simulink model "WT_FFNN_trainbfg_15_15_15_Dec_22_RepFast"  (R2021a)
settings: Solver=FixedStepAuto  StartTime=0  StopTime=T  FixedStep=Ts  RelTol=1e-3  EnableMultiTasking=on
undefined symbols (not defined in the file): patch_sig, safe_patch_sig, sw
libraries: neural x50, simulink x3
(part 2 of 2)

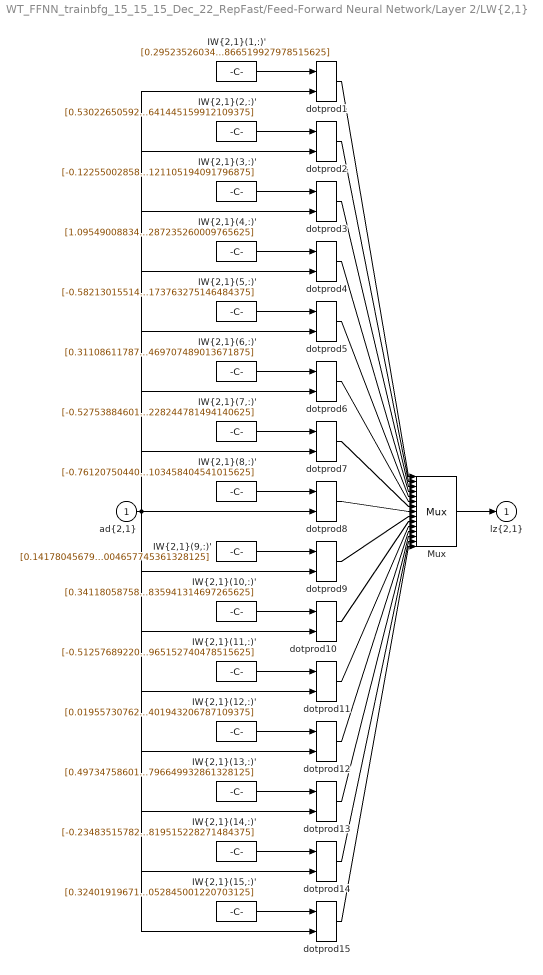
== system WT_FFNN_trainbfg_15_15_15_Dec_22_RepFast/Feed-Forward Neural Network/Layer 2/LW{2,1} ==
  "ad{2,1}" : Inport  PortDimensions=15
      mask Display: e = 0.06;c1 = [120 230 180]/255;c2 = ([120 230 180]+0)/(256+128);c3 = ([120 230 180]+128)/(256+128);patch([0 1 1 0],[0 0 1 1],c1);patch([0 1 1 1-e 1-e 0+e],[0 0 1 1-e 0+e 0+e],c2);patch([0 0 1 1-e 0+e 0+e],[0 1 1 1-e 1-e 0+e],c3);plot([0 1 1 0 0],[0 0 1 1 0]);
  "IW{2,1}(1,:)'" : Constant  Value=[0.295235260345368732970428027329035103321075439453125;-0.1676828200604070229218223175848834216594696044921875;0.089432221053525662313177235773764550685882568359375;0.54396077110849017088867185520939528942108154296875;-0.30457465744494971460198939894326031208038330078125;-0.96084475289336257475270031136460602283477783203125;0.5808144359338267559422774866106919944286346435546875;-0.1860903257221864226522711760480888187885284423828125;0.7014253485780148622552587767131626605987548828125;-0.54431412858791627940036050858907401561737060546875;0.5380581706717924017624454791075550019741058349609375;-0.9009348419158775822523921306128613650798797607421875;-0.7521354448038597428904949993011541664600372314453125;0.241917287870616615208518851432017982006072998046875;-0.7321374980240575869316899115801788866519927978515625]
      mask Display: e = 0.06;c1 = [120 150 230]/255;c2 = ([120 150 230]+0)/383;c3 = ([120 150 230]+128)/383;patch([0 1 1 0],[0 0 1 1],c1);patch([0 1 1 1-e 1-e 0+e],[0 0 1 1-e 0+e 0+e],c2);patch([0 0 1 1-e 0+e 0+e],[0 1 1 1-e 1-e 0+e],c3);plot([0 1 1 0 0],[0 0 1 1 0]);disp('weights');
  "IW{2,1}(10,:)'" : Constant  Value=[0.3411805875894959871885703250882215797901153564453125;-0.36412192595956416329983085233834572136402130126953125;-0.64636339290746036567725241184234619140625;0.722279622786664798894662453676573932170867919921875;-0.27904982791519883367215015823603607714176177978515625;0.68360886979400292684516671215533278882503509521484375;0.97808482860116885415635579192894510924816131591796875;0.6199190595393042624294821507646702229976654052734375;0.72843908277886437740988867517444305121898651123046875;-0.83326035111029117530279108905233442783355712890625;-0.58147330032467425819930895158904604613780975341796875;-0.30410030612850647013800653439830057322978973388671875;-0.58836623426168210837516880928887985646724700927734375;0.968838908437390955441514961421489715576171875;0.68377280483594038429373540566302835941314697265625]
      mask Display: e = 0.06;c1 = [120 150 230]/255;c2 = ([120 150 230]+0)/383;c3 = ([120 150 230]+128)/383;patch([0 1 1 0],[0 0 1 1],c1);patch([0 1 1 1-e 1-e 0+e],[0 0 1 1-e 0+e 0+e],c2);patch([0 0 1 1-e 0+e 0+e],[0 1 1 1-e 1-e 0+e],c3);plot([0 1 1 0 0],[0 0 1 1 0]);disp('weights');
  "IW{2,1}(11,:)'" : Constant  Value=[-0.512576892202383671559573485865257680416107177734375;-0.64166672849162242897591568180359899997711181640625;-0.2323014726512367678079584720762795768678188323974609375;-0.004885732283956631914756396639631930156610906124114990234375;0.66589137226295747051807438765536062419414520263671875;-0.2068744392450924396431588547784485854208469390869140625;0.055562400254155118461962814535581856034696102142333984375;-0.0276621328029923348179597297757936757989227771759033203125;0.22700116851777263349276836379431188106536865234375;0.381837877655510082863798970720381475985050201416015625;0.373687162446426024420276235105120576918125152587890625;0.10188044464799216048955798896713531576097011566162109375;0.928861560137871578035628772340714931488037109375;0.83619474780461811036502695060335099697113037109375;0.42233175405663969659286749447346664965152740478515625]
      mask Display: e = 0.06;c1 = [120 150 230]/255;c2 = ([120 150 230]+0)/383;c3 = ([120 150 230]+128)/383;patch([0 1 1 0],[0 0 1 1],c1);patch([0 1 1 1-e 1-e 0+e],[0 0 1 1-e 0+e 0+e],c2);patch([0 0 1 1-e 0+e 0+e],[0 1 1 1-e 1-e 0+e],c3);plot([0 1 1 0 0],[0 0 1 1 0]);disp('weights');
  "IW{2,1}(12,:)'" : Constant  Value=[0.0195573076253098519783346631584208807907998561859130859375;0.96877950329973661069971058168448507785797119140625;-0.43906894185078815251443984379875473678112030029296875;-0.2453583760887959874796848680489347316324710845947265625;-0.429912780674979233541677103858091868460178375244140625;0.454767949982676278342097475615446455776691436767578125;0.612974659896225571031891377060674130916595458984375;-0.784699422493088771801694747409783303737640380859375;0.97821339088929182281617613625712692737579345703125;0.422244862396419839978278787384624592959880828857421875;0.1638567334025056165813793995766900479793548583984375;0.1225489164995739732599844273863709531724452972412109375;-0.7051550721363504248273557095672003924846649169921875;0.39408876509436707724631787641556002199649810791015625;0.712830466285756525479655465460382401943206787109375]
      mask Display: e = 0.06;c1 = [120 150 230]/255;c2 = ([120 150 230]+0)/383;c3 = ([120 150 230]+128)/383;patch([0 1 1 0],[0 0 1 1],c1);patch([0 1 1 1-e 1-e 0+e],[0 0 1 1-e 0+e 0+e],c2);patch([0 0 1 1-e 0+e 0+e],[0 1 1 1-e 1-e 0+e],c3);plot([0 1 1 0 0],[0 0 1 1 0]);disp('weights');
  "IW{2,1}(13,:)'" : Constant  Value=[0.49734758601192741167551503167487680912017822265625;0.456087717212201482208655534122954122722148895263671875;-0.354850716647025776762092164062778465449810028076171875;0.370056821822693116086355757943238131701946258544921875;0.35945755073370933008192196211894042789936065673828125;0.403962590618102412864942607484408654272556304931640625;0.2812584438426630750740287112421356141567230224609375;0.01267604058140091478901201327289527398534119129180908203125;0.0501638531721098901439148676217882893979549407958984375;0.66191317537370519819006631223601289093494415283203125;-0.819786337588402691523015164420939981937408447265625;-0.0870564870349785635550432516538421623408794403076171875;-0.77059092798831418935634474109974689781665802001953125;0.06492564894049072943271738722614827565848827362060546875;-0.31005397435624815205557069930364377796649932861328125]
      mask Display: e = 0.06;c1 = [120 150 230]/255;c2 = ([120 150 230]+0)/383;c3 = ([120 150 230]+128)/383;patch([0 1 1 0],[0 0 1 1],c1);patch([0 1 1 1-e 1-e 0+e],[0 0 1 1-e 0+e 0+e],c2);patch([0 0 1 1-e 0+e 0+e],[0 1 1 1-e 1-e 0+e],c3);plot([0 1 1 0 0],[0 0 1 1 0]);disp('weights');
  "IW{2,1}(14,:)'" : Constant  Value=[-0.2348351578285707841331486633862368762493133544921875;-0.064245850300208129368684240034781396389007568359375;0.6412050242524041099301257418119348585605621337890625;0.483055790205989155072785479205776937305927276611328125;0.400497833477529485701751355009037069976329803466796875;-0.245029018628923456191159857553429901599884033203125;-0.69720340711643780107209522611810825765132904052734375;-0.70745219481255927629348434493294917047023773193359375;-0.040138572521909075818680179281727760098874568939208984375;0.78407918172274826407175396525417454540729522705078125;0.242397800141408048535396346778725273907184600830078125;0.07763798805447734430185136034197057597339153289794921875;-0.7345468453233909844612981032696552574634552001953125;-0.54799275931600222033779346020310185849666595458984375;-0.09452344436802194438396185205419897101819515228271484375]
      mask Display: e = 0.06;c1 = [120 150 230]/255;c2 = ([120 150 230]+0)/383;c3 = ([120 150 230]+128)/383;patch([0 1 1 0],[0 0 1 1],c1);patch([0 1 1 1-e 1-e 0+e],[0 0 1 1-e 0+e 0+e],c2);patch([0 0 1 1-e 0+e 0+e],[0 1 1 1-e 1-e 0+e],c3);plot([0 1 1 0 0],[0 0 1 1 0]);disp('weights');
  "IW{2,1}(15,:)'" : Constant  Value=[0.32401919671826906466094442293979227542877197265625;0.27772538922407574712991618071100674569606781005859375;0.25589672598047841223234399876673705875873565673828125;0.03997845702521808652907253645025775767862796783447265625;-0.116249832056752155917678237528889440000057220458984375;-0.56796216807721133790209933067671954631805419921875;-0.60041201485130313297844395492575131356716156005859375;-0.890051706187623636878925026394426822662353515625;0.60263542093203981142579550578375346958637237548828125;0.963512604604961353516046074219048023223876953125;-0.276048475872037124556612752712680958211421966552734375;-0.1097733012448873779476343770511448383331298828125;-0.66715673418933019167553766237688250839710235595703125;-0.2029144931375184424116042691821348853409290313720703125;-0.8924339193614028165058016384136863052845001220703125]
      mask Display: e = 0.06;c1 = [120 150 230]/255;c2 = ([120 150 230]+0)/383;c3 = ([120 150 230]+128)/383;patch([0 1 1 0],[0 0 1 1],c1);patch([0 1 1 1-e 1-e 0+e],[0 0 1 1-e 0+e 0+e],c2);patch([0 0 1 1-e 0+e 0+e],[0 1 1 1-e 1-e 0+e],c3);plot([0 1 1 0 0],[0 0 1 1 0]);disp('weights');
  "IW{2,1}(2,:)'" : Constant  Value=[0.5302265059205459873936661097104661166667938232421875;0.56475845138696723068960636737756431102752685546875;0.289664279816221614805016315585817210376262664794921875;0.8636390282028738596409311867319047451019287109375;-0.83362192000415868964324772605323232710361480712890625;-0.32183369212487911159570330710266716778278350830078125;0.75628015692548478110524001749581657350063323974609375;0.50230327800125673665121439626091159880161285400390625;0.11937217688658485759134464387898333370685577392578125;-0.09668324036885701799892700591954053379595279693603515625;-0.046385487394211201428451118999873870052397251129150390625;0.044395647902648216476251263884478248655796051025390625;-0.00954028462260186373156134465034483582712709903717041015625;0.03576122102860723739325976566760800778865814208984375;-1.087387383095764104012914685881696641445159912109375]
      mask Display: e = 0.06;c1 = [120 150 230]/255;c2 = ([120 150 230]+0)/383;c3 = ([120 150 230]+128)/383;patch([0 1 1 0],[0 0 1 1],c1);patch([0 1 1 1-e 1-e 0+e],[0 0 1 1-e 0+e 0+e],c2);patch([0 0 1 1-e 0+e 0+e],[0 1 1 1-e 1-e 0+e],c3);plot([0 1 1 0 0],[0 0 1 1 0]);disp('weights');
  "IW{2,1}(3,:)'" : Constant  Value=[-0.122550028588137294160986812130431644618511199951171875;0.8040681415155563893648604789632372558116912841796875;0.0700803874628591894069273848799639381468296051025390625;0.86939028804827123142473510597483254969120025634765625;0.412087729344845887791137784006423316895961761474609375;-0.29275208488329063083455139349098317325115203857421875;-0.421436955168346505384846523156738840043544769287109375;0.40171474062549805683630665953387506306171417236328125;0.86673742143877918753247513450332917273044586181640625;0.7464565387159451947951538386405445635318756103515625;0.77358975929442330699004060079460032284259796142578125;-0.74128481048777583595210671774111688137054443359375;1.0107702803741853703201059033744968473911285400390625;-1.015420261737861817863404212403111159801483154296875;0.99610375682476604008996901029604487121105194091796875]
      mask Display: e = 0.06;c1 = [120 150 230]/255;c2 = ([120 150 230]+0)/383;c3 = ([120 150 230]+128)/383;patch([0 1 1 0],[0 0 1 1],c1);patch([0 1 1 1-e 1-e 0+e],[0 0 1 1-e 0+e 0+e],c2);patch([0 0 1 1-e 0+e 0+e],[0 1 1 1-e 1-e 0+e],c3);plot([0 1 1 0 0],[0 0 1 1 0]);disp('weights');
  "IW{2,1}(4,:)'" : Constant  Value=[1.0954900883453830839897591431508772075176239013671875;-1.0671398314434192844402105038170702755451202392578125;0.4674545926284678909468084384570829570293426513671875;-0.622334117614310233790320125990547239780426025390625;-0.50044651341551193990397905508871190249919891357421875;-0.41617167669077270719668604215257801115512847900390625;0.554605315996658188026913194335065782070159912109375;0.68495334159006715513129393002600409090518951416015625;0.380392781972371418763856354416930116713047027587890625;-0.403210535716429119279524684316129423677921295166015625;0.0996010326827965475349202506549772806465625762939453125;-0.55362973136024018483425379599793814122676849365234375;0.76341803366177474199361085993587039411067962646484375;0.75787617513104288402558950110687874257564544677734375;-0.63575117538482450729730999228195287287235260009765625]
      mask Display: e = 0.06;c1 = [120 150 230]/255;c2 = ([120 150 230]+0)/383;c3 = ([120 150 230]+128)/383;patch([0 1 1 0],[0 0 1 1],c1);patch([0 1 1 1-e 1-e 0+e],[0 0 1 1-e 0+e 0+e],c2);patch([0 0 1 1-e 0+e 0+e],[0 1 1 1-e 1-e 0+e],c3);plot([0 1 1 0 0],[0 0 1 1 0]);disp('weights');
  "IW{2,1}(5,:)'" : Constant  Value=[-0.582130155147954297945034340955317020416259765625;0.226921473625750547142843061010353267192840576171875;0.0449906115542042517319032413070090115070343017578125;-0.7222515943416893957618185595492832362651824951171875;-0.9110918154435230231769082820392213761806488037109375;-0.6058924038090884867102658972726203501224517822265625;-0.122710034826088776327424056944437325000762939453125;-0.3629515092020156874497160970349796116352081298828125;0.165581930351680117752266596653498709201812744140625;0.6903563701080732695203323601162992417812347412109375;-0.96603412332547744512112330994568765163421630859375;-0.5890116581846402965538800344802439212799072265625;-0.45941133541460477118789640371687710285186767578125;0.457323363356542333946208600536920130252838134765625;-0.408932331049287167701322687207721173763275146484375]
      mask Display: e = 0.06;c1 = [120 150 230]/255;c2 = ([120 150 230]+0)/383;c3 = ([120 150 230]+128)/383;patch([0 1 1 0],[0 0 1 1],c1);patch([0 1 1 1-e 1-e 0+e],[0 0 1 1-e 0+e 0+e],c2);patch([0 0 1 1-e 0+e 0+e],[0 1 1 1-e 1-e 0+e],c3);plot([0 1 1 0 0],[0 0 1 1 0]);disp('weights');
  "IW{2,1}(6,:)'" : Constant  Value=[0.3110861178764547929631589795462787151336669921875;-0.538125541393581929838774158270098268985748291015625;1.0922620681325267977257453821948729455471038818359375;0.47206045307648636377706452549318782985210418701171875;0.406596366182418955670385685152723453938961029052734375;0.64098472753113833189075876362039707601070404052734375;0.69478739666693722920598474956932477653026580810546875;0.054751583517420716884505083044132334180176258087158203125;0.62813081168441431412219344565528444945812225341796875;-0.2061992856573582333368221952696330845355987548828125;-0.85292749069341422529788587780785746872425079345703125;-0.64614216631411014457597730142879299819469451904296875;-0.705984380169617953271199439768679440021514892578125;0.70665367079108165615508596602012403309345245361328125;-0.52734700314943949717161331136594526469707489013671875]
      mask Display: e = 0.06;c1 = [120 150 230]/255;c2 = ([120 150 230]+0)/383;c3 = ([120 150 230]+128)/383;patch([0 1 1 0],[0 0 1 1],c1);patch([0 1 1 1-e 1-e 0+e],[0 0 1 1-e 0+e 0+e],c2);patch([0 0 1 1-e 0+e 0+e],[0 1 1 1-e 1-e 0+e],c3);plot([0 1 1 0 0],[0 0 1 1 0]);disp('weights');
  "IW{2,1}(7,:)'" : Constant  Value=[-0.5275388460124068590317847338155843317508697509765625;0.63968120217193635834718179467017762362957000732421875;-1.4284826471654101798236524700769223272800445556640625;-0.87089994099444234532114705871208570897579193115234375;-0.727791167771064895219979007379151880741119384765625;-0.140157181233467209580112466937862336635589599609375;0.36231999642735213118527326514595188200473785400390625;-0.82009864245883790090374532155692577362060546875;0.75357372007314304962477535809739492833614349365234375;0.6501208183024740350219872198067605495452880859375;0.722174859333458929455673569464124739170074462890625;-0.78697167378918475577620483818463981151580810546875;0.469890026516892100882927252314402721822261810302734375;-1.1508080217275782342056800189311616122722625732421875;0.2368252313630880012684798430200316943228244781494140625]
      mask Display: e = 0.06;c1 = [120 150 230]/255;c2 = ([120 150 230]+0)/383;c3 = ([120 150 230]+128)/383;patch([0 1 1 0],[0 0 1 1],c1);patch([0 1 1 1-e 1-e 0+e],[0 0 1 1-e 0+e 0+e],c2);patch([0 0 1 1-e 0+e 0+e],[0 1 1 1-e 1-e 0+e],c3);plot([0 1 1 0 0],[0 0 1 1 0]);disp('weights');
  "IW{2,1}(8,:)'" : Constant  Value=[-0.7612075044053889794071210417314432561397552490234375;0.90690656912513512022400163914426229894161224365234375;-0.85143144253750058236818176737870089709758758544921875;0.04780801927375631643624132038894458673894405364990234375;-0.1744673941545842599243343329362687654793262481689453125;0.7755419085127075451424616403528489172458648681640625;-0.67686592553680269279681169791729189455509185791015625;-0.776588511613593102111963162315078079700469970703125;0.97930676436914365634578416575095616281032562255859375;-0.265526583954380723806565356426290236413478851318359375;-0.0072625998806437851162964847162584192119538784027099609375;-0.93420966482242018269488426085445098578929901123046875;0.1878646683548915452544036952531314454972743988037109375;0.7518711623440605951174120491486974060535430908203125;0.266611480614983575865295506446273066103458404541015625]
      mask Display: e = 0.06;c1 = [120 150 230]/255;c2 = ([120 150 230]+0)/383;c3 = ([120 150 230]+128)/383;patch([0 1 1 0],[0 0 1 1],c1);patch([0 1 1 1-e 1-e 0+e],[0 0 1 1-e 0+e 0+e],c2);patch([0 0 1 1-e 0+e 0+e],[0 1 1 1-e 1-e 0+e],c3);plot([0 1 1 0 0],[0 0 1 1 0]);disp('weights');
  "IW{2,1}(9,:)'" : Constant  Value=[0.1417804567956018058083600408281199634075164794921875;-0.69552074345356695861397611224674619734287261962890625;-0.8666039658670074974367025788524188101291656494140625;-0.01732820083515733411427817145522567443549633026123046875;0.2389862039024584217106195183077943511307239532470703125;-0.236256188189785609754522965886280871927738189697265625;0.63365984517294438038703674465068615972995758056640625;-0.76292736525968740668446343988762237131595611572265625;-1.0008999859346239258428568064118735492229461669921875;0.056428107179615917543546999013415188528597354888916015625;0.4593302753053769560409591576899401843547821044921875;0.2149457557622795611518284886187757365405559539794921875;-0.056642227092704888757879189142840914428234100341796875;0.63895629042777668527008927412680350244045257568359375;-1.008264007948838969497273865272291004657745361328125]
      mask Display: e = 0.06;c1 = [120 150 230]/255;c2 = ([120 150 230]+0)/383;c3 = ([120 150 230]+128)/383;patch([0 1 1 0],[0 0 1 1],c1);patch([0 1 1 1-e 1-e 0+e],[0 0 1 1-e 0+e 0+e],c2);patch([0 0 1 1-e 0+e 0+e],[0 1 1 1-e 1-e 0+e],c3);plot([0 1 1 0 0],[0 0 1 1 0]);disp('weights');
  Mux : Mux  Inputs=15
      mask Display: e = 0.06;c1 = [120 150 230]/255;c2 = ([120 150 230]+0)/383;c3 = ([120 150 230]+128)/383;patch([0 1 1 0],[0 0 1 1],c1);patch([0 1 1 1-e 1-e 0+e],[0 0 1 1-e 0+e 0+e],c2);patch([0 0 1 1-e 0+e 0+e],[0 1 1 1-e 1-e 0+e],c3);plot([0 1 1 0 0],[0 0 1 1 0]);disp('Mux');
  dotprod{1..15} (15 alike) : neural/Weight Functions/dotprod
  "lz{2,1}" : Outport
      mask Display: e = 0.06;c1 = [120 230 180]/255;c2 = ([120 230 180]+0)/(256+128);c3 = ([120 230 180]+128)/(256+128);patch([0 1 1 0],[0 0 1 1],c1);patch([0 1 1 1-e 1-e 0+e],[0 0 1 1-e 0+e 0+e],c2);patch([0 0 1 1-e 0+e 0+e],[0 1 1 1-e 1-e 0+e],c3);plot([0 1 1 0 0],[0 0 1 1 0]);
  wires:
  "IW{2,1}(1,:)'"/1 -> dotprod1/1
  "ad{2,1}"/1 -> dotprod1/2, dotprod2/2, dotprod3/2, dotprod4/2, dotprod5/2, dotprod6/2, dotprod7/2, dotprod8/2, dotprod9/2, dotprod10/2, dotprod11/2, dotprod12/2, dotprod13/2, dotprod14/2, dotprod15/2
  dotprod1/1 -> Mux/1
  "IW{2,1}(2,:)'"/1 -> dotprod2/1
  dotprod2/1 -> Mux/2
  "IW{2,1}(3,:)'"/1 -> dotprod3/1
  dotprod3/1 -> Mux/3
  "IW{2,1}(4,:)'"/1 -> dotprod4/1
  dotprod4/1 -> Mux/4
  "IW{2,1}(5,:)'"/1 -> dotprod5/1
  dotprod5/1 -> Mux/5
  "IW{2,1}(6,:)'"/1 -> dotprod6/1
  dotprod6/1 -> Mux/6
  "IW{2,1}(7,:)'"/1 -> dotprod7/1
  dotprod7/1 -> Mux/7
  "IW{2,1}(8,:)'"/1 -> dotprod8/1
  dotprod8/1 -> Mux/8
  "IW{2,1}(9,:)'"/1 -> dotprod9/1
  dotprod9/1 -> Mux/9
  "IW{2,1}(10,:)'"/1 -> dotprod10/1
  dotprod10/1 -> Mux/10
  "IW{2,1}(11,:)'"/1 -> dotprod11/1
  dotprod11/1 -> Mux/11
  "IW{2,1}(12,:)'"/1 -> dotprod12/1
  dotprod12/1 -> Mux/12
  "IW{2,1}(13,:)'"/1 -> dotprod13/1
  dotprod13/1 -> Mux/13
  "IW{2,1}(14,:)'"/1 -> dotprod14/1
  dotprod14/1 -> Mux/14
  "IW{2,1}(15,:)'"/1 -> dotprod15/1
  dotprod15/1 -> Mux/15
  Mux/1 -> "lz{2,1}"/1

== system WT_FFNN_trainbfg_15_15_15_Dec_22_RepFast/Feed-Forward Neural Network/Layer 3/Delays 1 ==
  "p{3}" : Inport  PortDimensions=15
      mask Display: e = 0.06;c1 = [120 230 180]/255;c2 = ([120 230 180]+0)/(256+128);c3 = ([120 230 180]+128)/(256+128);patch([0 1 1 0],[0 0 1 1],c1);patch([0 1 1 1-e 1-e 0+e],[0 0 1 1-e 0+e 0+e],c2);patch([0 0 1 1-e 0+e 0+e],[0 1 1 1-e 1-e 0+e],c3);plot([0 1 1 0 0],[0 0 1 1 0]);
  mux : Mux  Inputs=1
      mask Display: e = 0.06;c1 = [120 150 230]/255;c2 = ([120 150 230]+0)/383;c3 = ([120 150 230]+128)/383;patch([0 1 1 0],[0 0 1 1],c1);patch([0 1 1 1-e 1-e 0+e],[0 0 1 1-e 0+e 0+e],c2);patch([0 0 1 1-e 0+e 0+e],[0 1 1 1-e 1-e 0+e],c3);plot([0 1 1 0 0],[0 0 1 1 0]);disp('Mux')
  "pd{3,2}" : Outport
      mask Display: e = 0.06;c1 = [120 230 180]/255;c2 = ([120 230 180]+0)/(256+128);c3 = ([120 230 180]+128)/(256+128);patch([0 1 1 0],[0 0 1 1],c1);patch([0 1 1 1-e 1-e 0+e],[0 0 1 1-e 0+e 0+e],c2);patch([0 0 1 1-e 0+e 0+e],[0 1 1 1-e 1-e 0+e],c3);plot([0 1 1 0 0],[0 0 1 1 0]);
  wires:
  "p{3}"/1 -> mux/1
  mux/1 -> "pd{3,2}"/1

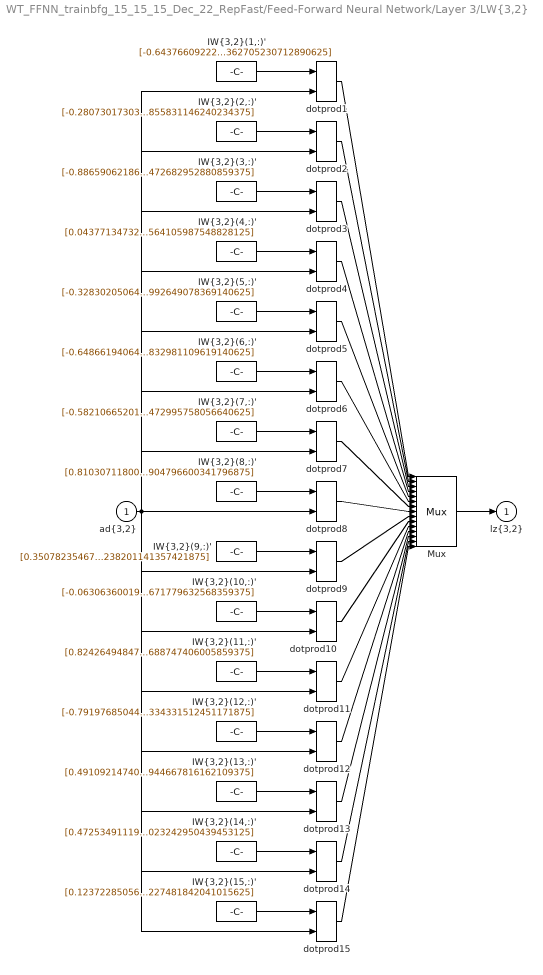
== system WT_FFNN_trainbfg_15_15_15_Dec_22_RepFast/Feed-Forward Neural Network/Layer 3/LW{3,2} ==
  "ad{3,2}" : Inport  PortDimensions=15
      mask Display: e = 0.06;c1 = [120 230 180]/255;c2 = ([120 230 180]+0)/(256+128);c3 = ([120 230 180]+128)/(256+128);patch([0 1 1 0],[0 0 1 1],c1);patch([0 1 1 1-e 1-e 0+e],[0 0 1 1-e 0+e 0+e],c2);patch([0 0 1 1-e 0+e 0+e],[0 1 1 1-e 1-e 0+e],c3);plot([0 1 1 0 0],[0 0 1 1 0]);
  "IW{3,2}(1,:)'" : Constant  Value=[-0.643766092226467190329231016221456229686737060546875;-0.63161180496894697711240951321087777614593505859375;-0.0878846663125170124430951545946300029754638671875;0.0675439035340004156893201070488430559635162353515625;0.3850639727730376105085952076478861272335052490234375;-0.897336227775257899708094555535353720188140869140625;0.4800646559755552544856982422061264514923095703125;-0.5886509570704803184781894742627628147602081298828125;-0.7754320756879466980393544872640632092952728271484375;-0.0247924491321527273868241536547429859638214111328125;-0.81529532256159686909313677460886538028717041015625;-0.367142001707418064171406513196416199207305908203125;0.9758694699049907939070180873386561870574951171875;-0.2984465102282147785928145822254009544849395751953125;-0.750254482560374302835271009826101362705230712890625]
      mask Display: e = 0.06;c1 = [120 150 230]/255;c2 = ([120 150 230]+0)/383;c3 = ([120 150 230]+128)/383;patch([0 1 1 0],[0 0 1 1],c1);patch([0 1 1 1-e 1-e 0+e],[0 0 1 1-e 0+e 0+e],c2);patch([0 0 1 1-e 0+e 0+e],[0 1 1 1-e 1-e 0+e],c3);plot([0 1 1 0 0],[0 0 1 1 0]);disp('weights');
  "IW{3,2}(10,:)'" : Constant  Value=[-0.0630636001920052979841102569480426609516143798828125;-0.138562076770683939574979604003601707518100738525390625;0.5037893785023583870241736804018728435039520263671875;-0.37852129015125601796398768783546984195709228515625;-0.7442232404340096696415685073588974773883819580078125;-1.5274447744213108801858425067621283233165740966796875;0.47475882919923584335464283867622725665569305419921875;-0.51218928545745889824303276327555067837238311767578125;0.046979185094962967739196102456844528205692768096923828125;-0.89472131757113115835267080910853110253810882568359375;-0.67996225419660649702535692995297722518444061279296875;0.665075343023343368287214616429992020130157470703125;0.155923146673057455569022522468003444373607635498046875;-0.41606152437333132620977949045482091605663299560546875;0.52807136530591092249409257419756613671779632568359375]
      mask Display: e = 0.06;c1 = [120 150 230]/255;c2 = ([120 150 230]+0)/383;c3 = ([120 150 230]+128)/383;patch([0 1 1 0],[0 0 1 1],c1);patch([0 1 1 1-e 1-e 0+e],[0 0 1 1-e 0+e 0+e],c2);patch([0 0 1 1-e 0+e 0+e],[0 1 1 1-e 1-e 0+e],c3);plot([0 1 1 0 0],[0 0 1 1 0]);disp('weights');
  "IW{3,2}(11,:)'" : Constant  Value=[0.82426494847924569597807931131683290004730224609375;-0.97790085353089961639483362887403927743434906005859375;0.05798050134246912623581238221959210932254791259765625;0.0522049315911223832387122456566430628299713134765625;0.0990802140303959077982653980143368244171142578125;0.22106217246656834074514108579023741185665130615234375;0.5494379678203917816148305064416490495204925537109375;-0.5531961288794098319243630612618289887905120849609375;-0.85830145284077807854572483847732655704021453857421875;-0.3683771233222679075680616733734495937824249267578125;-0.84421218908653639090289289015345275402069091796875;0.228393991214632274822093904731445945799350738525390625;-0.6995068658844585396394677445641718804836273193359375;-0.329454009632487221370666929942672140896320343017578125;0.51859940161120388069093678495846688747406005859375]
      mask Display: e = 0.06;c1 = [120 150 230]/255;c2 = ([120 150 230]+0)/383;c3 = ([120 150 230]+128)/383;patch([0 1 1 0],[0 0 1 1],c1);patch([0 1 1 1-e 1-e 0+e],[0 0 1 1-e 0+e 0+e],c2);patch([0 0 1 1-e 0+e 0+e],[0 1 1 1-e 1-e 0+e],c3);plot([0 1 1 0 0],[0 0 1 1 0]);disp('weights');
  "IW{3,2}(12,:)'" : Constant  Value=[-0.7919768504412429965810815701843239367008209228515625;1.0033848061042613952764668283634819090366363525390625;-1.0390198514651327599267460755072534084320068359375;0.49160142077057711329501898944727145135402679443359375;-0.029541182830081336163630112423561513423919677734375;-0.306332999843011266616343846180825494229793548583984375;-0.28816981566130428493721638005808927118778228759765625;-0.004029605993336768214596599335663995589129626750946044921875;0.83117708491185948727064669583342038094997406005859375;0.69780510277171725608269525764626450836658477783203125;-0.75061795071970838222341626533307135105133056640625;-0.026106209111428212155114891857010661624372005462646484375;-0.01326470024297421966552601446664994000457227230072021484375;0.028940856769380872426378203954300261102616786956787109375;0.48065458023885454519330551192979328334331512451171875]
      mask Display: e = 0.06;c1 = [120 150 230]/255;c2 = ([120 150 230]+0)/383;c3 = ([120 150 230]+128)/383;patch([0 1 1 0],[0 0 1 1],c1);patch([0 1 1 1-e 1-e 0+e],[0 0 1 1-e 0+e 0+e],c2);patch([0 0 1 1-e 0+e 0+e],[0 1 1 1-e 1-e 0+e],c3);plot([0 1 1 0 0],[0 0 1 1 0]);disp('weights');
  "IW{3,2}(13,:)'" : Constant  Value=[0.4910921474034346534409678497468121349811553955078125;-0.35340206811983032597623832771205343306064605712890625;-1.176008886905686612323052031570114195346832275390625;0.418378994498182610328740338445641100406646728515625;0.7809513583688765248069785229745320975780487060546875;0.23836109638957603262809925581677816808223724365234375;-0.5879442809896107124956188272335566580295562744140625;-0.81700253732117555927061403053812682628631591796875;-0.70337928386330006436111261791666038334369659423828125;0.4279767684318735998516558538540266454219818115234375;-0.94735904487062783108086705396999605000019073486328125;-0.372677364151523082824724042438901960849761962890625;-0.55839089993002366529850633014575578272342681884765625;0.31116974169516320447570478791021741926670074462890625;0.4873766829746519757549094720161519944667816162109375]
      mask Display: e = 0.06;c1 = [120 150 230]/255;c2 = ([120 150 230]+0)/383;c3 = ([120 150 230]+128)/383;patch([0 1 1 0],[0 0 1 1],c1);patch([0 1 1 1-e 1-e 0+e],[0 0 1 1-e 0+e 0+e],c2);patch([0 0 1 1-e 0+e 0+e],[0 1 1 1-e 1-e 0+e],c3);plot([0 1 1 0 0],[0 0 1 1 0]);disp('weights');
  "IW{3,2}(14,:)'" : Constant  Value=[0.4725349111932770629351807656348682940006256103515625;-0.64786214511093376255956854947726242244243621826171875;0.38324798288263017820298728111083619296550750732421875;0.715268424425147930634238946367986500263214111328125;0.597920557625758686270955877262167632579803466796875;0.5038424204816511764448705434915609657764434814453125;-1.6304705087709490118896837884676642715930938720703125;-0.05343899095897287898626615287867025472223758697509765625;-0.1289058344562188096471544440646539442241191864013671875;-0.56593574312072736365308855965849943459033966064453125;-0.34810180729696160728536824535694904625415802001953125;-0.89576670443147354827573280999786220490932464599609375;0.70614267092802140979301839252002537250518798828125;-0.32965131765960420384686813122243620455265045166015625;-0.78815891360858547631806914068874903023242950439453125]
      mask Display: e = 0.06;c1 = [120 150 230]/255;c2 = ([120 150 230]+0)/383;c3 = ([120 150 230]+128)/383;patch([0 1 1 0],[0 0 1 1],c1);patch([0 1 1 1-e 1-e 0+e],[0 0 1 1-e 0+e 0+e],c2);patch([0 0 1 1-e 0+e 0+e],[0 1 1 1-e 1-e 0+e],c3);plot([0 1 1 0 0],[0 0 1 1 0]);disp('weights');
  "IW{3,2}(15,:)'" : Constant  Value=[0.12372285056327481100879595032893121242523193359375;-0.417466162302169319087141730051371268928050994873046875;0.74889684910740739187673398191691376268863677978515625;-1.2419287871508177811818995905923657119274139404296875;0.4686821673919394637408686321577988564968109130859375;-0.9028301562390428358639837824739515781402587890625;0.94328518915823489354721687050187028944492340087890625;-0.8868517157212674195676527233445085585117340087890625;0.200793237968276805371914406350697390735149383544921875;-0.75836216632250808000748065751395188271999359130859375;-0.35716046908971044171465791805530898272991180419921875;0.125342530379980221511004856438376009464263916015625;0.61567850861981454624327625424484722316265106201171875;-0.54471415826170643814663208104320801794528961181640625;0.36349890803543927209062758265645243227481842041015625]
      mask Display: e = 0.06;c1 = [120 150 230]/255;c2 = ([120 150 230]+0)/383;c3 = ([120 150 230]+128)/383;patch([0 1 1 0],[0 0 1 1],c1);patch([0 1 1 1-e 1-e 0+e],[0 0 1 1-e 0+e 0+e],c2);patch([0 0 1 1-e 0+e 0+e],[0 1 1 1-e 1-e 0+e],c3);plot([0 1 1 0 0],[0 0 1 1 0]);disp('weights');
  "IW{3,2}(2,:)'" : Constant  Value=[-0.2807301730358393587749787911889143288135528564453125;0.19442270067570976976867314078845083713531494140625;-0.7966612127504897333807321047061122953891754150390625;-0.7816915759150828701962154809734784066677093505859375;0.1133396699280251329611246546846814453601837158203125;-0.854229401802047760838831891305744647979736328125;-0.530346170504191416483763532596640288829803466796875;-0.2234567379043965740237354111741296947002410888671875;0.5688557814878254514923128226655535399913787841796875;0.5379165281177382684774102017399854958057403564453125;-0.9843594128613302185470956828794442117214202880859375;-0.564873381154358700229067835607565939426422119140625;-0.6591359538862333611319854753674007952213287353515625;0.3710714174950744403957969552720896899700164794921875;-0.951131967899252028786349910660646855831146240234375]
      mask Display: e = 0.06;c1 = [120 150 230]/255;c2 = ([120 150 230]+0)/383;c3 = ([120 150 230]+128)/383;patch([0 1 1 0],[0 0 1 1],c1);patch([0 1 1 1-e 1-e 0+e],[0 0 1 1-e 0+e 0+e],c2);patch([0 0 1 1-e 0+e 0+e],[0 1 1 1-e 1-e 0+e],c3);plot([0 1 1 0 0],[0 0 1 1 0]);disp('weights');
  "IW{3,2}(3,:)'" : Constant  Value=[-0.8865906218634176383375233854167163372039794921875;-0.448077337715563406295160575609770603477954864501953125;0.913293669289934495481020348961465060710906982421875;0.0243638308880861249872129548066368442960083484649658203125;-0.20695841483681487460444259340874850749969482421875;-1.2133496936065666371717952642939053475856781005859375;0.9142109435884802071115018406999297440052032470703125;-0.0704803471330011921391900386879569850862026214599609375;-0.6365282917209567070671027977368794381618499755859375;-0.232690998135838655880291980793117545545101165771484375;0.053595784013774593057544137764125480316579341888427734375;-0.60642288792672882635770292836241424083709716796875;-0.457989591376957327906183081722701899707317352294921875;-0.56406227387336560497033133287914097309112548828125;-0.419649478389224339647256556418142281472682952880859375]
      mask Display: e = 0.06;c1 = [120 150 230]/255;c2 = ([120 150 230]+0)/383;c3 = ([120 150 230]+128)/383;patch([0 1 1 0],[0 0 1 1],c1);patch([0 1 1 1-e 1-e 0+e],[0 0 1 1-e 0+e 0+e],c2);patch([0 0 1 1-e 0+e 0+e],[0 1 1 1-e 1-e 0+e],c3);plot([0 1 1 0 0],[0 0 1 1 0]);disp('weights');
  "IW{3,2}(4,:)'" : Constant  Value=[0.0437713473225584959180878286133520305156707763671875;-0.76778442161840343427314792279503308236598968505859375;-0.39661496563128884051963041201815940439701080322265625;-0.386674253628728592513397188668022863566875457763671875;-0.8768186658920706921804821831756271421909332275390625;0.463302794105690141091002942630439065396785736083984375;0.92038779657970282155332597540109418332576751708984375;-0.5261575263558324611068428566795773804187774658203125;0.1583872574595577564782189483594265766441822052001953125;-0.45393034172955870619858842474059201776981353759765625;0.259495472072293564824718714589835144579410552978515625;0.76346444985456984877458808114170096814632415771484375;-0.2007035972545312685344498504491639323532581329345703125;-0.0110954620547697550836385715911092120222747325897216796875;-0.3650038428544306601253310873289592564105987548828125]
      mask Display: e = 0.06;c1 = [120 150 230]/255;c2 = ([120 150 230]+0)/383;c3 = ([120 150 230]+128)/383;patch([0 1 1 0],[0 0 1 1],c1);patch([0 1 1 1-e 1-e 0+e],[0 0 1 1-e 0+e 0+e],c2);patch([0 0 1 1-e 0+e 0+e],[0 1 1 1-e 1-e 0+e],c3);plot([0 1 1 0 0],[0 0 1 1 0]);disp('weights');
  "IW{3,2}(5,:)'" : Constant  Value=[-0.3283020506461509224749306667945347726345062255859375;-0.63368807272042315670290690832189284265041351318359375;-0.50004509247909301183909747123834677040576934814453125;-0.53062901555559383037774523472762666642665863037109375;0.5603510629823471589361361111514270305633544921875;0.6472426878442194553286981317796744406223297119140625;0.80879347157413350455357203827588818967342376708984375;0.1813632071858231054051202590926550328731536865234375;0.85475663679927560423266186262480914592742919921875;-0.925564320323100542253769162925891578197479248046875;0.6106125056115214722041173445177264511585235595703125;0.07253728678965991327753926043442334048449993133544921875;-0.912406020826254771094454554258845746517181396484375;0.59384277518434347431508513182052411139011383056640625;0.307601515186365137566326666274107992649078369140625]
      mask Display: e = 0.06;c1 = [120 150 230]/255;c2 = ([120 150 230]+0)/383;c3 = ([120 150 230]+128)/383;patch([0 1 1 0],[0 0 1 1],c1);patch([0 1 1 1-e 1-e 0+e],[0 0 1 1-e 0+e 0+e],c2);patch([0 0 1 1-e 0+e 0+e],[0 1 1 1-e 1-e 0+e],c3);plot([0 1 1 0 0],[0 0 1 1 0]);disp('weights');
  "IW{3,2}(6,:)'" : Constant  Value=[-0.6486619406486784367160680631059221923351287841796875;0.82867439648848095767874610828584991395473480224609375;-0.99191269994009889643393762526102364063262939453125;0.430265984839494686209349083583219908177852630615234375;-0.3248322718959097965552018649759702384471893310546875;0.281955136991089594378223637249902822077274322509765625;-0.82759268769953553412932478750008158385753631591796875;-0.03135210614543824936273352932403213344514369964599609375;-0.151764941130526020973690037862979806959629058837890625;0.39320585006210617695643350089085288345813751220703125;0.017800096072113184841878563702266546897590160369873046875;0.09175282271876682160804961085887043736875057220458984375;0.3626375185956021152122730200062505900859832763671875;0.11652429763007328411550389546391670592129230499267578125;0.91387076939331779446007431033649481832981109619140625]
      mask Display: e = 0.06;c1 = [120 150 230]/255;c2 = ([120 150 230]+0)/383;c3 = ([120 150 230]+128)/383;patch([0 1 1 0],[0 0 1 1],c1);patch([0 1 1 1-e 1-e 0+e],[0 0 1 1-e 0+e 0+e],c2);patch([0 0 1 1-e 0+e 0+e],[0 1 1 1-e 1-e 0+e],c3);plot([0 1 1 0 0],[0 0 1 1 0]);disp('weights');
  "IW{3,2}(7,:)'" : Constant  Value=[-0.582106652013729242156614418490789830684661865234375;-0.8570943744259109653427231023670174181461334228515625;-0.40351205622447228194005219847895205020904541015625;-0.979326763313207226957501916331239044666290283203125;0.215731814525891518741218533250503242015838623046875;-0.735834088572874467359952177503146231174468994140625;-0.2671267673616022353400012434576638042926788330078125;-0.6963089497674668226778749158256687223911285400390625;0.3895043892358802661846084447461180388927459716796875;-0.14087108149629390396739836432971060276031494140625;-0.782364123453909154903840317274443805217742919921875;-0.631132664484693517437108312151394784450531005859375;-0.19522333460767615775921512977220118045806884765625;-0.3293773385895077954188536750734783709049224853515625;0.8714617455697608594533676296123303472995758056640625]
      mask Display: e = 0.06;c1 = [120 150 230]/255;c2 = ([120 150 230]+0)/383;c3 = ([120 150 230]+128)/383;patch([0 1 1 0],[0 0 1 1],c1);patch([0 1 1 1-e 1-e 0+e],[0 0 1 1-e 0+e 0+e],c2);patch([0 0 1 1-e 0+e 0+e],[0 1 1 1-e 1-e 0+e],c3);plot([0 1 1 0 0],[0 0 1 1 0]);disp('weights');
  "IW{3,2}(8,:)'" : Constant  Value=[0.8103071180089280733938039702479727566242218017578125;-0.54024673189444361032229835473117418587207794189453125;-0.91108785616791643224843255666201002895832061767578125;-0.981283640646074761804129593656398355960845947265625;0.4825080990044359197099765879102051258087158203125;0.343603815709114190912742969885584898293018341064453125;-0.261603910195804256755280903234961442649364471435546875;0.5638641465853277967568146777921356260776519775390625;0.4790134717783678386382462122128345072269439697265625;-0.0968789693578998301060067888101912103593349456787109375;0.253615987989335989194472631425014697015285491943359375;-0.59677651927548847066162807095679454505443572998046875;0.9229100859841417037188193717156536877155303955078125;-0.4304415853880516618090723568457178771495819091796875;-0.084227332291266332475743183749727904796600341796875]
      mask Display: e = 0.06;c1 = [120 150 230]/255;c2 = ([120 150 230]+0)/383;c3 = ([120 150 230]+128)/383;patch([0 1 1 0],[0 0 1 1],c1);patch([0 1 1 1-e 1-e 0+e],[0 0 1 1-e 0+e 0+e],c2);patch([0 0 1 1-e 0+e 0+e],[0 1 1 1-e 1-e 0+e],c3);plot([0 1 1 0 0],[0 0 1 1 0]);disp('weights');
  "IW{3,2}(9,:)'" : Constant  Value=[0.35078235467249374579523646389134228229522705078125;-0.892491215582572383624437861726619303226470947265625;0.010856284915405911561947505106218159198760986328125;0.3358322431472473557079183592577464878559112548828125;-0.7903735160530007686219278184580616652965545654296875;-0.7792930387153027549373973670299164950847625732421875;0.3700569453232185335167514494969509541988372802734375;-0.7987873552751569850016721829888410866260528564453125;-0.1347153477057989601206600127625279128551483154296875;0.2197143385804321003007544277352280914783477783203125;-0.7470002693413941852185189418378286063671112060546875;-0.8453063837746463971001276149763725697994232177734375;-0.195632029555030673151350129046477377414703369140625;-0.0948149168613519055526239753817208111286163330078125;-0.5190432063358307868128349582548253238201141357421875]
      mask Display: e = 0.06;c1 = [120 150 230]/255;c2 = ([120 150 230]+0)/383;c3 = ([120 150 230]+128)/383;patch([0 1 1 0],[0 0 1 1],c1);patch([0 1 1 1-e 1-e 0+e],[0 0 1 1-e 0+e 0+e],c2);patch([0 0 1 1-e 0+e 0+e],[0 1 1 1-e 1-e 0+e],c3);plot([0 1 1 0 0],[0 0 1 1 0]);disp('weights');
  Mux : Mux  Inputs=15
      mask Display: e = 0.06;c1 = [120 150 230]/255;c2 = ([120 150 230]+0)/383;c3 = ([120 150 230]+128)/383;patch([0 1 1 0],[0 0 1 1],c1);patch([0 1 1 1-e 1-e 0+e],[0 0 1 1-e 0+e 0+e],c2);patch([0 0 1 1-e 0+e 0+e],[0 1 1 1-e 1-e 0+e],c3);plot([0 1 1 0 0],[0 0 1 1 0]);disp('Mux');
  dotprod{1..15} (15 alike) : neural/Weight Functions/dotprod
  "lz{3,2}" : Outport
      mask Display: e = 0.06;c1 = [120 230 180]/255;c2 = ([120 230 180]+0)/(256+128);c3 = ([120 230 180]+128)/(256+128);patch([0 1 1 0],[0 0 1 1],c1);patch([0 1 1 1-e 1-e 0+e],[0 0 1 1-e 0+e 0+e],c2);patch([0 0 1 1-e 0+e 0+e],[0 1 1 1-e 1-e 0+e],c3);plot([0 1 1 0 0],[0 0 1 1 0]);
  wires:
  "IW{3,2}(1,:)'"/1 -> dotprod1/1
  "ad{3,2}"/1 -> dotprod1/2, dotprod2/2, dotprod3/2, dotprod4/2, dotprod5/2, dotprod6/2, dotprod7/2, dotprod8/2, dotprod9/2, dotprod10/2, dotprod11/2, dotprod12/2, dotprod13/2, dotprod14/2, dotprod15/2
  dotprod1/1 -> Mux/1
  "IW{3,2}(2,:)'"/1 -> dotprod2/1
  dotprod2/1 -> Mux/2
  "IW{3,2}(3,:)'"/1 -> dotprod3/1
  dotprod3/1 -> Mux/3
  "IW{3,2}(4,:)'"/1 -> dotprod4/1
  dotprod4/1 -> Mux/4
  "IW{3,2}(5,:)'"/1 -> dotprod5/1
  dotprod5/1 -> Mux/5
  "IW{3,2}(6,:)'"/1 -> dotprod6/1
  dotprod6/1 -> Mux/6
  "IW{3,2}(7,:)'"/1 -> dotprod7/1
  dotprod7/1 -> Mux/7
  "IW{3,2}(8,:)'"/1 -> dotprod8/1
  dotprod8/1 -> Mux/8
  "IW{3,2}(9,:)'"/1 -> dotprod9/1
  dotprod9/1 -> Mux/9
  "IW{3,2}(10,:)'"/1 -> dotprod10/1
  dotprod10/1 -> Mux/10
  "IW{3,2}(11,:)'"/1 -> dotprod11/1
  dotprod11/1 -> Mux/11
  "IW{3,2}(12,:)'"/1 -> dotprod12/1
  dotprod12/1 -> Mux/12
  "IW{3,2}(13,:)'"/1 -> dotprod13/1
  dotprod13/1 -> Mux/13
  "IW{3,2}(14,:)'"/1 -> dotprod14/1
  dotprod14/1 -> Mux/14
  "IW{3,2}(15,:)'"/1 -> dotprod15/1
  dotprod15/1 -> Mux/15
  Mux/1 -> "lz{3,2}"/1

== system WT_FFNN_trainbfg_15_15_15_Dec_22_RepFast/Feed-Forward Neural Network/Layer 4/Delays 1 ==
  "p{4}" : Inport  PortDimensions=15
      mask Display: e = 0.06;c1 = [120 230 180]/255;c2 = ([120 230 180]+0)/(256+128);c3 = ([120 230 180]+128)/(256+128);patch([0 1 1 0],[0 0 1 1],c1);patch([0 1 1 1-e 1-e 0+e],[0 0 1 1-e 0+e 0+e],c2);patch([0 0 1 1-e 0+e 0+e],[0 1 1 1-e 1-e 0+e],c3);plot([0 1 1 0 0],[0 0 1 1 0]);
  mux : Mux  Inputs=1
      mask Display: e = 0.06;c1 = [120 150 230]/255;c2 = ([120 150 230]+0)/383;c3 = ([120 150 230]+128)/383;patch([0 1 1 0],[0 0 1 1],c1);patch([0 1 1 1-e 1-e 0+e],[0 0 1 1-e 0+e 0+e],c2);patch([0 0 1 1-e 0+e 0+e],[0 1 1 1-e 1-e 0+e],c3);plot([0 1 1 0 0],[0 0 1 1 0]);disp('Mux')
  "pd{4,3}" : Outport
      mask Display: e = 0.06;c1 = [120 230 180]/255;c2 = ([120 230 180]+0)/(256+128);c3 = ([120 230 180]+128)/(256+128);patch([0 1 1 0],[0 0 1 1],c1);patch([0 1 1 1-e 1-e 0+e],[0 0 1 1-e 0+e 0+e],c2);patch([0 0 1 1-e 0+e 0+e],[0 1 1 1-e 1-e 0+e],c3);plot([0 1 1 0 0],[0 0 1 1 0]);
  wires:
  "p{4}"/1 -> mux/1
  mux/1 -> "pd{4,3}"/1

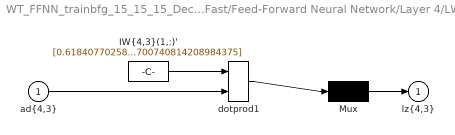
== system WT_FFNN_trainbfg_15_15_15_Dec_22_RepFast/Feed-Forward Neural Network/Layer 4/LW{4,3} ==
  "ad{4,3}" : Inport  PortDimensions=15
      mask Display: e = 0.06;c1 = [120 230 180]/255;c2 = ([120 230 180]+0)/(256+128);c3 = ([120 230 180]+128)/(256+128);patch([0 1 1 0],[0 0 1 1],c1);patch([0 1 1 1-e 1-e 0+e],[0 0 1 1-e 0+e 0+e],c2);patch([0 0 1 1-e 0+e 0+e],[0 1 1 1-e 1-e 0+e],c3);plot([0 1 1 0 0],[0 0 1 1 0]);
  "IW{4,3}(1,:)'" : Constant  Value=[0.61840770258758670507859278586693108081817626953125;0.4972377435523942512674011595663614571094512939453125;-0.527033565992718333603761493577621877193450927734375;-0.11604922719461170654842163685316336341202259063720703125;-0.289333266477987682829819959806627593934535980224609375;0.5076960079193586494739065528847277164459228515625;-0.20223849523360204472055556834675371646881103515625;0.07883746407795717836552995549936895258724689483642578125;-0.63852447949041124530822344240732491016387939453125;-0.9976873501248981757072442633216269314289093017578125;-0.942546450600823870757949407561682164669036865234375;0.6257132065110564411725135869346559047698974609375;0.5590218477028316979016153709380887448787689208984375;1.1391616199309384516169529888429678976535797119140625;-1.1781364434347894043497717575519345700740814208984375]
      mask Display: e = 0.06;c1 = [120 150 230]/255;c2 = ([120 150 230]+0)/383;c3 = ([120 150 230]+128)/383;patch([0 1 1 0],[0 0 1 1],c1);patch([0 1 1 1-e 1-e 0+e],[0 0 1 1-e 0+e 0+e],c2);patch([0 0 1 1-e 0+e 0+e],[0 1 1 1-e 1-e 0+e],c3);plot([0 1 1 0 0],[0 0 1 1 0]);disp('weights');
  Mux : Mux  Inputs=1
      mask Display: e = 0.06;c1 = [120 150 230]/255;c2 = ([120 150 230]+0)/383;c3 = ([120 150 230]+128)/383;patch([0 1 1 0],[0 0 1 1],c1);patch([0 1 1 1-e 1-e 0+e],[0 0 1 1-e 0+e 0+e],c2);patch([0 0 1 1-e 0+e 0+e],[0 1 1 1-e 1-e 0+e],c3);plot([0 1 1 0 0],[0 0 1 1 0]);disp('Mux');
  dotprod1 : neural/Weight Functions/dotprod
  "lz{4,3}" : Outport
      mask Display: e = 0.06;c1 = [120 230 180]/255;c2 = ([120 230 180]+0)/(256+128);c3 = ([120 230 180]+128)/(256+128);patch([0 1 1 0],[0 0 1 1],c1);patch([0 1 1 1-e 1-e 0+e],[0 0 1 1-e 0+e 0+e],c2);patch([0 0 1 1-e 0+e 0+e],[0 1 1 1-e 1-e 0+e],c3);plot([0 1 1 0 0],[0 0 1 1 0]);
  wires:
  "IW{4,3}(1,:)'"/1 -> dotprod1/1
  "ad{4,3}"/1 -> dotprod1/2
  dotprod1/1 -> Mux/1
  Mux/1 -> "lz{4,3}"/1
